simulink model "compute_ud_sim"  (Simulink 4.00)
settings: Solver=ode45  StartTime=0.0  StopTime=10.0  RelTol=1e-3
values from neighbouring files (symbols this model uses):
  P = Phi*P*Phi' + Q    [covanal.m]
undefined symbols (not defined in the file or in its folder): compute_d, compute_u
settings Model: Creator=mcar  LastModifiedBy=mcar  BlockReductionOpt=off

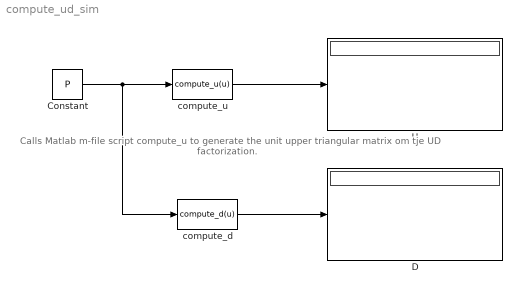
== system compute_ud_sim ==
  note: Calls Matlab m-file script compute_u
      | to generate the unit upper triangular
      | matrix om tje UD factorization.
  Constant : Constant  Value=P
  D : Display
      settings: Format=short
  U : Display
      settings: Format=short
  compute_d : MATLABFcn  MATLABFcn=compute_d(u)  OutputDimensions=-1  OutputSignalType=auto  Output1D=off
  compute_u : MATLABFcn  MATLABFcn=compute_u(u)  OutputDimensions=-1  OutputSignalType=auto  Output1D=off
  wires:
  Constant/1 -> compute_u/1, compute_d/1
  compute_u/1 -> U/1
  compute_d/1 -> D/1
